simulink model "ride_demo_quartercar"  (R2025b)
settings: Solver=ode4  StartTime=0.0  StopTime=numel(ride_speeds) * ride_dt  FixedStep=ride_dt_sim  RelTol=1e-3
InitFcn:
  | if isempty(which('ride.run'))
  |     run(fullfile(fileparts(get_param(bdroot, 'FileName')), '..', 'setup.m'));
  | end
  | if ~exist('ride_road', 'var') || ~exist('ride_speeds', 'var')
  |     ride_demo_run = ride.run(ride.config('model', 'quartercar'));
  |     ride_road = ride_demo_run.road;
  |     ride_speeds = ride_demo_run.speeds;
  |     ride_dt = ride_demo_run.P.DT;
  |     ride_dt_sim = ride_demo_run.P.DT_SIM;
  |     clear ride_demo_run
  | end
libraries: ride_lib x3
settings Model: Creator=mohammedazab  LastModifiedBy=mohammedazab
settings DataIOCC: SaveOutput=off  SaveTime=off

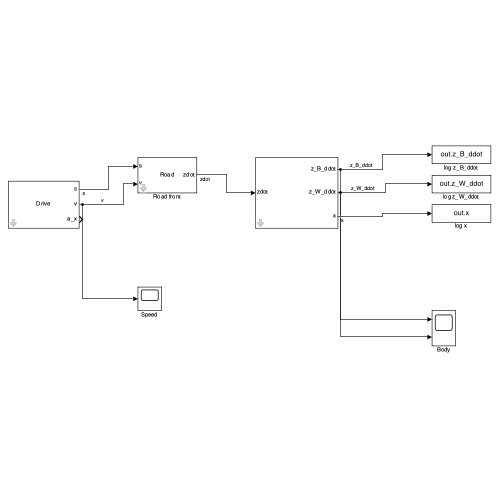
[thumbnail: Simulink's stored preview of the top-level diagram]
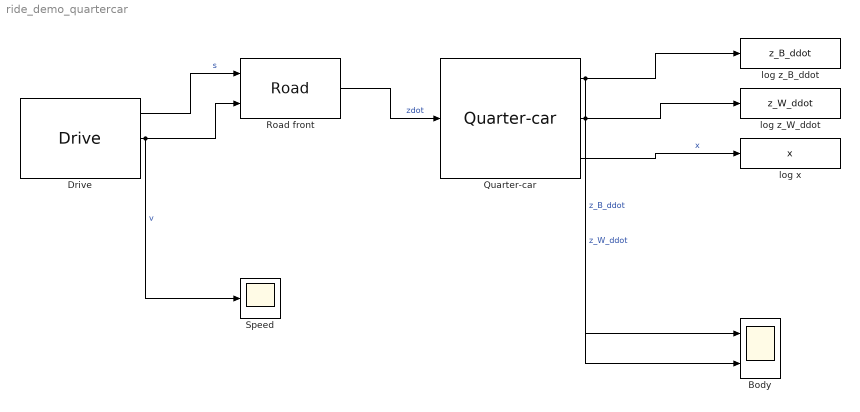
== system ride_demo_quartercar ==
  Body : Scope  NumInputPorts=2
  Drive : ride_lib/Drive  speeds=ride_speeds  dt=ride_dt
  Quarter-car : ride_lib/Quarter-car  m_B=465.69999999999999  m_W=50.399999999999999  k_T=262200  c_T=500  k_S=27922  dz_S_stat=0.16361711195473103  dz_cmp=0.02  dz_rbd=0.080000000000000002  f1_cmp=0.33333333329999998  f2_cmp=4  f1_rbd=1  f2_rbd=8  F_max=100000  D=3530  A=0.5  v_d=0.20000000000000001  v_z=0.20000000000000001
  Road front : ride_lib/Road  road=ride_road  lag_m=0
  Speed : Scope
  log x : ToWorkspace  VariableName=x  SampleTime=ride_dt
  log z_B_ddot : ToWorkspace  VariableName=z_B_ddot  SampleTime=ride_dt
  log z_W_ddot : ToWorkspace  VariableName=z_W_ddot  SampleTime=ride_dt
  wires:
  Drive/1 -> Road front/1  "s"
  Drive/2 -> Road front/2, Speed/1  "v"
  Road front/1 -> Quarter-car/1  "zdot"
  Quarter-car/1 -> log z_B_ddot/1, Body/1  "z_B_ddot"
  Quarter-car/2 -> log z_W_ddot/1, Body/2  "z_W_ddot"
  Quarter-car/3 -> log x/1  "x"
